simulink model "HW_Stepper_Motor"  (R2025b)
settings: Solver=FixedStepAuto  StartTime=0.0  StopTime=inf  FixedStep=0.05  RelTol=1e-3  EnableMultiTasking=on
libraries: raspberrypiBasiclib x7, simulink x1
settings Model: ExtModeTrigDuration=2  Creator=ioannisgeorgilas  LastModifiedBy=ioannisgeorgilas
settings SolverCC: PositivePriorityOrder=on
settings OptimizationCC: EnhancedBackFolding=on  PassReuseOutputArgsAs=Individual arguments  ZeroExternalMemoryAtStartup=off  ZeroInternalMemoryAtStartup=off  MaxStackSize=200000  OptimizeBlockOrder=speed  DifferentSizesBufferReuse=on  OptimizationCustomize=off  EfficientTunableParamExpr=on
settings DebuggingCC: ParameterTunabilityLossMsg=error
settings HardwareCC: ProdBitPerPointer=32.0  ProdBitPerSizeT=32.0  ProdBitPerPtrDiffT=32.0  ProdLargestAtomicInteger=Long  ProdLargestAtomicFloat=Double  ProdWordSize=32.0  ProdLongLongMode=on  ProdHWDeviceType=ARM Compatible->ARM Cortex-A (32-bit)
settings RTWCC: SystemTargetFile=ert.tlc  HardwareBoard=Raspberry Pi  TLCOptions="-aInlineSetEventsForThisBaseRateFcn=TLC_FALSE -aSuppressMultiTaskScheduler=TLC_FALSE  -aRateBasedStepFcn=0"  TemplateMakefile=ert_default_tmf  Toolchain=GNU GCC Embedded Linux  BuildConfiguration=Faster Runs  Description=Embedded Coder
settings CodeAppCC: ForceParamTrailComments=on  IgnoreCustomStorageClasses=off  OperatorAnnotations=on  SimulinkDataObjDesc=on  SFDataObjDesc=on  InsertBlockDesc=on
settings ERTTargetCC: ExtModeTransport=2.0  ExtModeStaticAlloc=on  ExtModeMexFile=ext_xcp  ExtModeIntrfLevel=Level2 - Open  InlinedParameterPlacement=Hierarchical  CodeReplacementLibrary=ARM Cortex-A CMSIS  SupportVariableSizeSignals=on

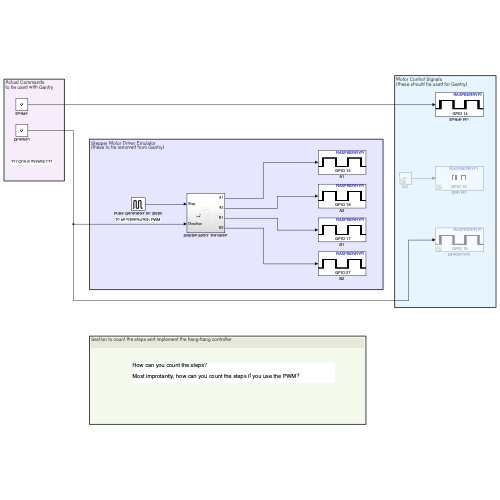
[thumbnail: Simulink's stored preview of the top-level diagram]
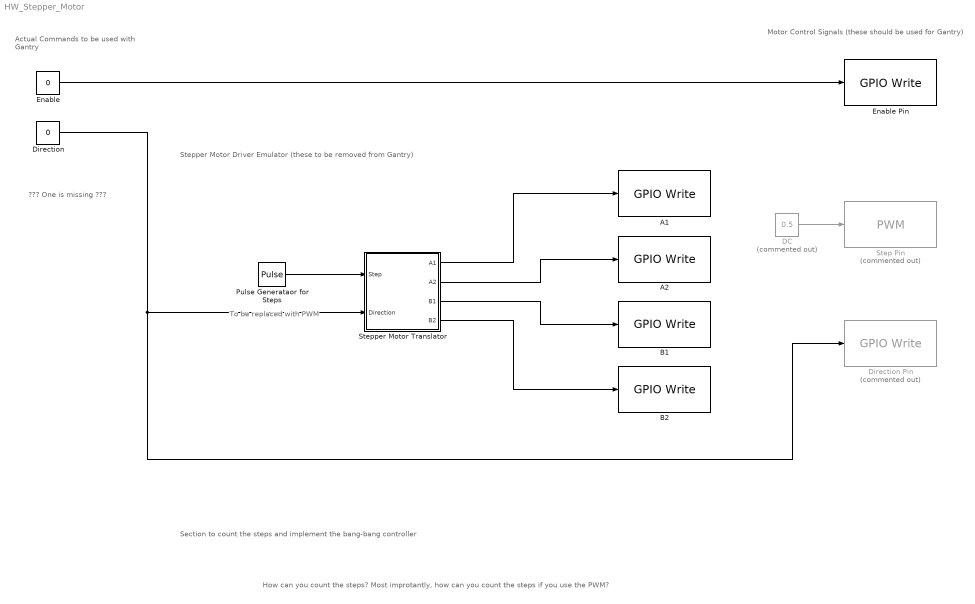
== system HW_Stepper_Motor ==
  note: Section to count the steps and implement the bang-bang controller
  note: ??? One is missing ???
  note: Actual Commands
      | to be used with Gantry
  note: To be replaced with PWM
  note: How can you count the steps?
      |
      | Most improtantly, how can you count the steps if you use the PWM?
  note: Motor Control Signals
      | (these should be used for Gantry)
  note: Stepper Motor Driver Emulator
      | (these to be removed from Gantry)
  A1 : raspberrypiBasiclib/GPIO Write  BoardProperty=Pi 3 Model B+  gpio=15  blockPlatform=Raspberry Pi  PinNumber=17  board=[]  direction=[]
  A2 : raspberrypiBasiclib/GPIO Write  BoardProperty=Pi 3 Model B+  gpio=18  blockPlatform=Raspberry Pi  PinNumber=17  board=[]  direction=[]
  B1 : raspberrypiBasiclib/GPIO Write  BoardProperty=Pi 3 Model B+  gpio=17  blockPlatform=Raspberry Pi  PinNumber=17  board=[]  direction=[]
  B2 : raspberrypiBasiclib/GPIO Write  BoardProperty=Pi 3 Model B+  gpio=27  blockPlatform=Raspberry Pi  PinNumber=17  board=[]  direction=[]
  DC : Constant  Commented=on  Value=0.5  SampleTime=-1
  Direction : Constant  Value=0  SampleTime=-1
  Direction Pin : raspberrypiBasiclib/GPIO Write  Commented=on  BoardProperty=Pi 3 Model B+  gpio=18  blockPlatform=Raspberry Pi  PinNumber=17  board=[]  direction=[]
  Enable : Constant  Value=0  SampleTime=-1
  Enable Pin : raspberrypiBasiclib/GPIO Write  BoardProperty=Pi 3 Model B+  gpio=14  blockPlatform=Raspberry Pi  PinNumber=17  board=[]  direction=[]
  Pulse Generataor for Steps : DiscretePulseGenerator  PulseType=Time based  Period=0.1  PulseWidth=50
  Step Pin : raspberrypiBasiclib/PWM  Commented=on  board=Pi 3 Model B+  Pin_=15  Frequency=100  blockPlatform=Raspberry Pi
  Stepper Motor Translator : Subsystem
  wires:
  Stepper Motor Translator/1(A1) -> A1/1
  Stepper Motor Translator/2(A2) -> A2/1
  Stepper Motor Translator/3(B1) -> B1/1
  Stepper Motor Translator/4(B2) -> B2/1
  Enable/1 -> Enable Pin/1
  Pulse Generataor for Steps/1 -> Stepper Motor Translator/1(Step)
  Direction/1 -> Direction Pin/1, Stepper Motor Translator/2(Direction)
  DC/1 -> Step Pin/1

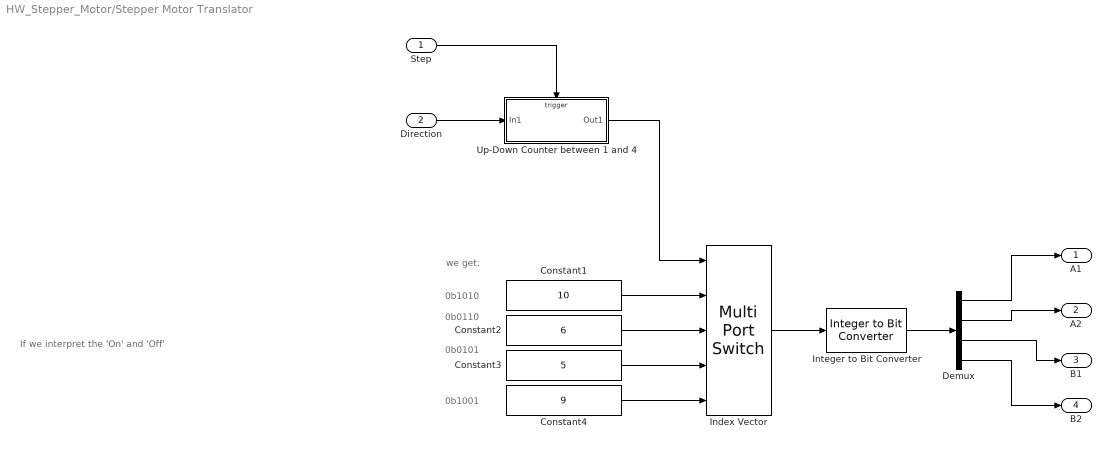
== system HW_Stepper_Motor/Stepper Motor Translator ==
  note: we get:
  note: If we interpret the 'On' and 'Off'
  note: 0b1010
  note: 0b0110
  note: 0b0101
  note: 0b1001
  Step : Inport
  Direction : Inport  Port=2
  Constant1 : Constant  Value=10  OutDataTypeStr=uint8  SampleTime=-1
  Constant2 : Constant  Value=6  OutDataTypeStr=uint8  SampleTime=-1
  Constant3 : Constant  Value=5  OutDataTypeStr=uint8  SampleTime=-1
  Constant4 : Constant  Value=9  OutDataTypeStr=uint8  SampleTime=-1
  Demux : Demux
  Index Vector : MultiPortSwitch  Inputs=4  SaturateOnIntegerOverflow=off  InputSameDT=off
  Integer to Bit Converter : simulink/Logic and Bit Operations/Integer to Bit Converter  nbits=4  signedInputValues=Unsigned  bitOrder=MSB first  outDtype=Inherit via internal rule
  Up-Down Counter between 1 and 4 : Subsystem  TreatAsAtomicUnit=on
  A1 : Outport
  A2 : Outport  Port=2
  B1 : Outport  Port=3
  B2 : Outport  Port=4
  wires:
  Demux/3 -> B1/1
  Index Vector/1 -> Integer to Bit Converter/1
  Constant3/1 -> Index Vector/4
  Demux/4 -> B2/1
  Demux/1 -> A1/1
  Up-Down Counter between 1 and 4/1(Out1) -> Index Vector/1
  Integer to Bit Converter/1 -> Demux/1
  Direction/1 -> Up-Down Counter between 1 and 4/1(In1)
  Demux/2 -> A2/1
  Constant1/1 -> Index Vector/2
  Constant2/1 -> Index Vector/3
  Step/1 -> Up-Down Counter between 1 and 4/Trigger
  Constant4/1 -> Index Vector/5

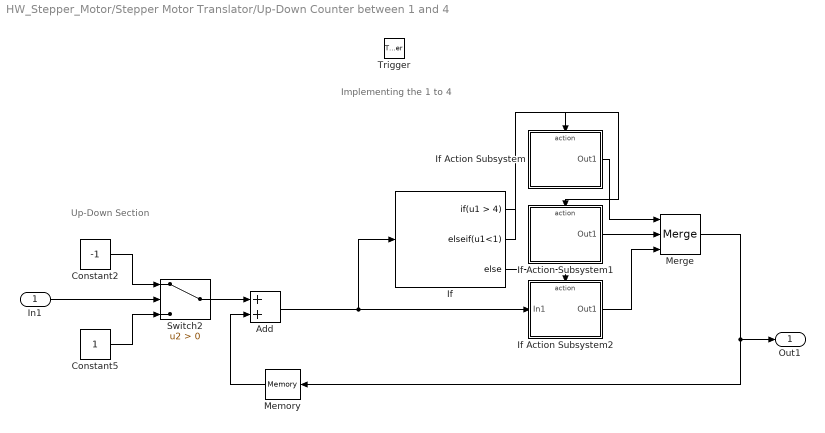
== system HW_Stepper_Motor/Stepper Motor Translator/Up-Down Counter between 1 and 4 ==
  note: Implementing the 1 to 4
  note: Up-Down Section
  In1 : Inport
  Trigger : TriggerPort  VariantControl=(inherit)  PortDimensions=1
  Add : Sum
  Constant2 : Constant  Value=-1  SampleTime=-1
  Constant5 : Constant  SampleTime=-1
  If : If  IfExpression=u1 > 4  ElseIfExpressions=u1<1
  If Action Subsystem : Subsystem  TreatAsAtomicUnit=on
  If Action Subsystem1 : Subsystem  TreatAsAtomicUnit=on
  If Action Subsystem2 : Subsystem  TreatAsAtomicUnit=on
  Memory : Memory  InitialCondition=1  InheritSampleTime=on
  Merge : Merge  Inputs=3
  Switch2 : Switch  Criteria=u2 > Threshold  SaturateOnIntegerOverflow=off  InputSameDT=off
  Out1 : Outport  InitialOutput=1
  wires:
  If Action Subsystem2/1(Out1) -> Merge/3
  If/2 -> If Action Subsystem1/Action
  If/3 -> If Action Subsystem2/Action
  Memory/1 -> Add/2
  Constant5/1 -> Switch2/3
  If/1 -> If Action Subsystem/Action
  If Action Subsystem1/1(Out1) -> Merge/2
  Constant2/1 -> Switch2/1
  Add/1 -> If/1, If Action Subsystem2/1(In1)
  If Action Subsystem/1(Out1) -> Merge/1
  Switch2/1 -> Add/1
  Merge/1 -> Memory/1, Out1/1
  In1/1 -> Switch2/2

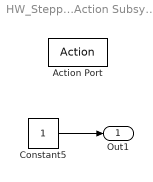
== system HW_Stepper_Motor/Stepper Motor Translator/Up-Down Counter between 1 and 4/If Action Subsystem ==
  Action Port : ActionPort  ActionPortLabel=if(u1 > 4)
  Constant5 : Constant  SampleTime=-1
  Out1 : Outport
  wires:
  Constant5/1 -> Out1/1

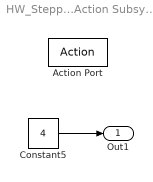
== system HW_Stepper_Motor/Stepper Motor Translator/Up-Down Counter between 1 and 4/If Action Subsystem1 ==
  Action Port : ActionPort  ActionPortLabel=elseif(u1<1)
  Constant5 : Constant  Value=4  SampleTime=-1
  Out1 : Outport
  wires:
  Constant5/1 -> Out1/1

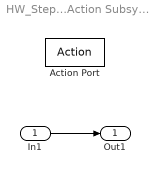
== system HW_Stepper_Motor/Stepper Motor Translator/Up-Down Counter between 1 and 4/If Action Subsystem2 ==
  In1 : Inport
  Action Port : ActionPort  ActionPortLabel=else
  Out1 : Outport
  wires:
  In1/1 -> Out1/1
